simulink model "lcc_plant"  (R2026b)
settings: Solver=ode4  StopTime=30  FixedStep=0.005
values from neighbouring files (symbols this model uses):
  P = lcc_plant_params("trailer")    [build_lcc_closed_loop.m]    (also in build_lcc_plant.m; lcc_scenario_input.m = lcc_plant_params(config); validate_lcc_plant.m)
undefined symbols (not defined in the file or in its folder): LANE
settings Model: Creator=kikiw  LastModifiedBy=kikiw
settings DebuggingCC: AlgebraicLoopMsg=error
settings ModelReferenceCC: ModelReferenceMinAlgLoopOccurrences=on

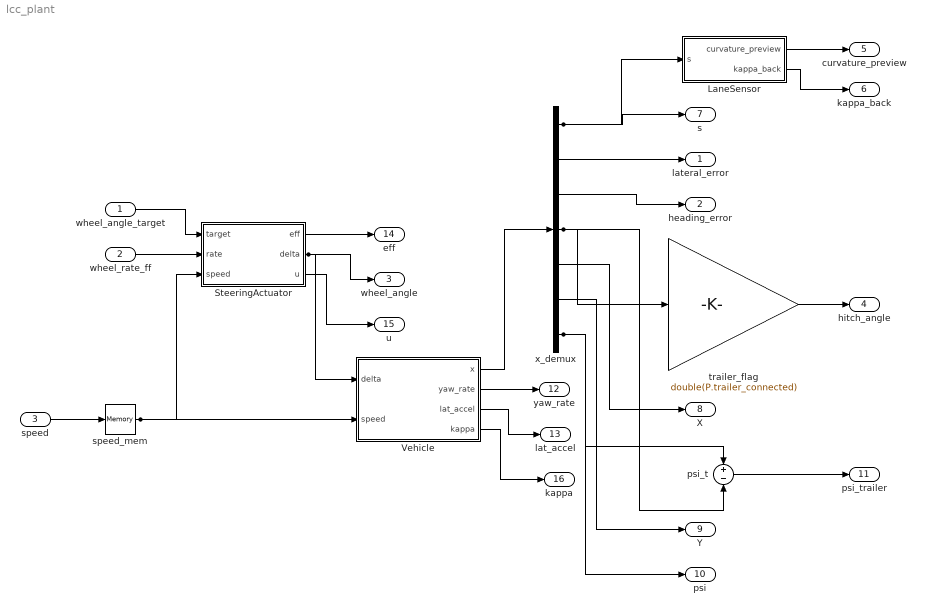
== system lcc_plant ==
  wheel_angle_target : Inport
  wheel_rate_ff : Inport  Port=2
  speed : Inport  Port=3
  LaneSensor : Subsystem
  SteeringActuator : Subsystem
  Vehicle : Subsystem
  psi_t : Sum  Inputs=+-
  speed_mem : Memory  InitialCondition=P.init.speed
  trailer_flag : Gain  Gain=double(P.trailer_connected)
  x_demux : Demux  Outputs=7
  lateral_error : Outport
  heading_error : Outport  Port=2
  wheel_angle : Outport  Port=3
  hitch_angle : Outport  Port=4
  curvature_preview : Outport  Port=5
  kappa_back : Outport  Port=6
  s : Outport  Port=7
  X : Outport  Port=8
  Y : Outport  Port=9
  psi : Outport  Port=10
  psi_trailer : Outport  Port=11
  yaw_rate : Outport  Port=12
  lat_accel : Outport  Port=13
  eff : Outport  Port=14
  u : Outport  Port=15
  kappa : Outport  Port=16
  wires:
  wheel_angle_target/1 -> SteeringActuator/1(target)
  speed_mem/1 -> Vehicle/2(speed), SteeringActuator/3(speed)
  speed/1 -> speed_mem/1
  wheel_rate_ff/1 -> SteeringActuator/2(rate)
  SteeringActuator/1(eff) -> eff/1
  x_demux/5 -> X/1
  SteeringActuator/2(delta) -> Vehicle/1(delta), wheel_angle/1
  SteeringActuator/3(u) -> u/1
  trailer_flag/1 -> hitch_angle/1
  Vehicle/1(x) -> x_demux/1
  Vehicle/2(yaw_rate) -> yaw_rate/1
  Vehicle/3(lat_accel) -> lat_accel/1
  Vehicle/4(kappa) -> kappa/1
  psi_t/1 -> psi_trailer/1
  x_demux/1 -> LaneSensor/1(s), s/1
  x_demux/2 -> lateral_error/1
  x_demux/3 -> heading_error/1
  x_demux/4 -> psi_t/2, trailer_flag/1
  x_demux/6 -> Y/1
  x_demux/7 -> psi_t/1, psi/1
  LaneSensor/1(curvature_preview) -> curvature_preview/1
  LaneSensor/2(kappa_back) -> kappa_back/1

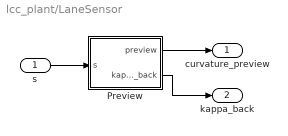
== system lcc_plant/LaneSensor ==
  s : Inport
  Preview : MATLAB Function  TreatAsAtomicUnit=on  SystemSampleTime=P.sim.ctrl_dt
  curvature_preview : Outport
  kappa_back : Outport  Port=2
  wires:
  s/1 -> Preview/1(s)
  Preview/1(preview) -> curvature_preview/1
  Preview/2(kappa_back) -> kappa_back/1

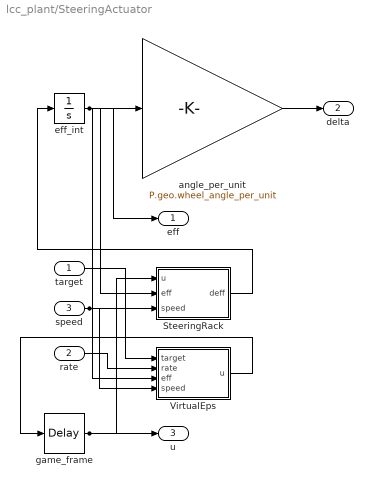
== system lcc_plant/SteeringActuator ==
  target : Inport
  rate : Inport  Port=2
  speed : Inport  Port=3
  SteeringRack : MATLAB Function  TreatAsAtomicUnit=on
  VirtualEps : MATLAB Function  TreatAsAtomicUnit=on  SystemSampleTime=P.sim.ctrl_dt
  angle_per_unit : Gain  Gain=P.geo.wheel_angle_per_unit
  eff_int : Integrator  InitialCondition=P.init.eff  LimitOutput=on  UpperSaturationLimit=P.geo.eff_max  LowerSaturationLimit=-P.geo.eff_max
  game_frame : TransportDelay  DelayTime=P.steer.delay
  eff : Outport
  delta : Outport  Port=2
  u : Outport  Port=3
  wires:
  angle_per_unit/1 -> delta/1
  eff_int/1 -> VirtualEps/3(eff), SteeringRack/2(eff), angle_per_unit/1, eff/1
  target/1 -> VirtualEps/1(target)
  speed/1 -> VirtualEps/4(speed), SteeringRack/3(speed)
  SteeringRack/1(deff) -> eff_int/1
  game_frame/1 -> SteeringRack/1(u), u/1
  rate/1 -> VirtualEps/2(rate)
  VirtualEps/1(u) -> game_frame/1

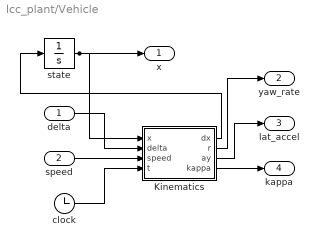
== system lcc_plant/Vehicle ==
  delta : Inport
  speed : Inport  Port=2
  Kinematics : MATLAB Function  TreatAsAtomicUnit=on
  clock : Clock
  state : Integrator  InitialCondition=[P.init.s; P.init.ey; P.init.epsi; P.init.hitch; P.init.X; P.init.Y; P.init.psi]
  x : Outport
  yaw_rate : Outport  Port=2
  lat_accel : Outport  Port=3
  kappa : Outport  Port=4
  wires:
  state/1 -> Kinematics/1(x), x/1
  Kinematics/4(kappa) -> kappa/1
  Kinematics/3(ay) -> lat_accel/1
  Kinematics/1(dx) -> state/1
  delta/1 -> Kinematics/2(delta)
  Kinematics/2(r) -> yaw_rate/1
  speed/1 -> Kinematics/3(speed)
  clock/1 -> Kinematics/4(t)

== matlab function lcc_plant/SteeringActuator/SteeringRack ==
  data: u input; deff output; eff input; speed input; P parameter
function deff = SteeringRack(u, eff, speed, P)
% measured relative steering: d(eff)/dt = a(v)*u - c(v)*eff (docs/31 조향 계통)
kmh = abs(speed) * 3.6;
a = interp1(P.steer.kmh, P.steer.a, min(kmh, P.steer.kmh(end)));
c = P.steer.c_scale * interp1(P.steer.kmh, P.steer.c, min(kmh, P.steer.kmh(end)));
deff = a * u - c * eff;

== matlab function lcc_plant/SteeringActuator/VirtualEps ==
  data: target input; u output; rate input; eff input; speed input; P parameter
function u = VirtualEps(target, rate, eff, speed, P)
% node inner loop (virtual_eps.hpp), 50 Hz
u = lcc_virtual_eps(target, rate, eff, speed, P.eps, P.geo.wheel_angle_per_unit);

== matlab function lcc_plant/Vehicle/Kinematics ==
  data: x input; dx output; delta input; speed input; t input; r output; ay output; kappa output; P parameter; LANE parameter
function [dx, r, ay, kappa] = Kinematics(x, delta, speed, t, P, LANE)
% x = [s; ey; epsi; hitch; X; Y; psi] (lcc_vehicle_deriv.m); slow yaw-rate wander P.dist
[~, kappa] = lcc_lane_lookup(LANE, x(1));
d = sum(P.dist.amp * sin(2*pi*P.dist.freq*t + P.dist.phase));
[dx, r, ay] = lcc_vehicle_deriv(x, delta, speed, P.geo.L, kappa, P, d);

== matlab function lcc_plant/LaneSensor/Preview ==
  data: s input; preview output; kappa_back output; P parameter; LANE parameter
function [preview, kappa_back] = Preview(s, P, LANE)
% node: LanePath::curvature(s + i*ds, window), i = 0..60
[preview, kappa_back] = lcc_lane_sensor(s, LANE, P.lane);
